simulink model "sine_fft_spectrum"  (R2026b)
settings: Solver=FixedStepDiscrete  StopTime=2  FixedStep=6.25e-05
PreLoadFcn:
  | addpath('C:\Users\jkung\Dropbox\proj\ClaudeCode\Matlab');
model workspace (MAT data in the model file):
  f_sig = 1000
settings Model: Creator=jkung  LastModifiedBy=jkung

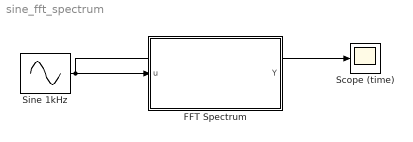
== system sine_fft_spectrum ==
  FFT Spectrum : MATLAB Function  TreatAsAtomicUnit=on
  Scope (time) : Scope
  Sine 1kHz : Sin  Frequency=2*pi*f_sig  SampleTime=6.25e-05
  wires:
  Sine 1kHz/1 -> Scope (time)/1, FFT Spectrum/1(u)

== matlab function sine_fft_spectrum/FFT Spectrum ==
  data: u input double size=1; Y output double size=[513 1]
function Y = fft_spectrum(u)
% Sliding 1024-sample buffer; a new spectrum is computed every N samples.
% Y: single-sided magnitude in dB (513 bins), 1 V sine peak -> 0 dB.
coder.extrinsic('show_spectrum');   % plot runs as plain MATLAB during simulation
N = 1024;
persistent buf cnt Ymag w
if isempty(buf)
    buf  = zeros(N,1);
    cnt  = 0;
    Ymag = -200*ones(N/2+1,1);
    w    = 0.5 - 0.5*cos(2*pi*(0:N-1)'/N);     % periodic Hann window
end
buf = [buf(2:end); u];
cnt = cnt + 1;
if cnt >= N
    cnt = 0;
    X   = fft(buf .* w);
    Ymag = 20*log10(abs(X(1:N/2+1)) * 2 / sum(w) + eps);
    show_spectrum(Ymag, 16000);          % live plot, once per FFT frame
end
Y = Ymag;
end
